simulink model "DIGITAL_WATCH_STAGE7"  (R2026b)
settings: Solver=VariableStepAuto  StopTime=3600
libraries: simulink_extras x21
settings Model: Creator=Trealer  LastModifiedBy=Trealer

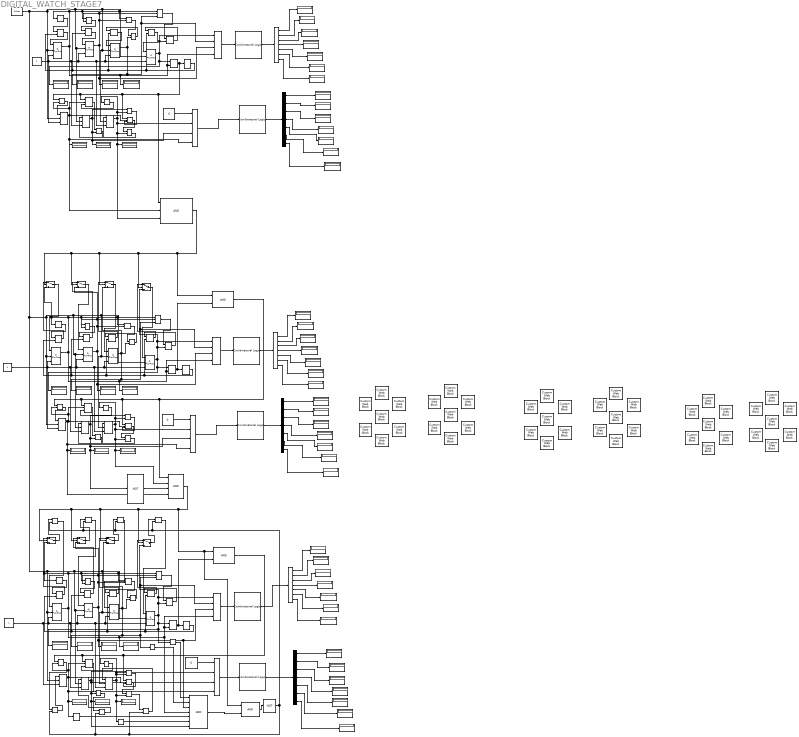
== system DIGITAL_WATCH_STAGE7 ==
  A{,1..5} (6 alike) : Display
  AND{,1..4,7..11,14,17..25} (20 alike) : Logic  IconShape=distinctive  AllPortsSameDT=off  OutDataTypeStr=boolean
  "AND-GATE MIN-EN " : Logic  Inputs=3  IconShape=distinctive  AllPortsSameDT=off  OutDataTypeStr=boolean
  AND-gate : Logic  IconShape=distinctive  AllPortsSameDT=off  OutDataTypeStr=boolean
  AND-gate1 : Logic  IconShape=distinctive  AllPortsSameDT=off  OutDataTypeStr=boolean
  AND-gate2 : Logic  Inputs=3  IconShape=distinctive  AllPortsSameDT=off  OutDataTypeStr=boolean
  AND-gate3 : Logic  Inputs=3  IconShape=distinctive  AllPortsSameDT=off  OutDataTypeStr=boolean
  AND-gate4 : Logic  IconShape=distinctive  AllPortsSameDT=off  OutDataTypeStr=boolean
  AND-gate5 : Logic  Inputs=3  IconShape=distinctive  AllPortsSameDT=off  OutDataTypeStr=boolean
  AND{5..6,12..13,15..16} (6 alike) : Logic  Inputs=3  IconShape=distinctive  AllPortsSameDT=off  OutDataTypeStr=boolean
  B{,1..5} (6 alike) : Display
  C{,1..5} (6 alike) : Display
  C_HR : Logic  IconShape=distinctive  AllPortsSameDT=off  OutDataTypeStr=boolean
  C_HU : Logic  IconShape=distinctive  AllPortsSameDT=off  OutDataTypeStr=boolean
  C_MIN : Logic  IconShape=distinctive  AllPortsSameDT=off  OutDataTypeStr=boolean
  C_MU : Logic  IconShape=distinctive  AllPortsSameDT=off  OutDataTypeStr=boolean
  Combinatorial Logic : CombinatorialLogic  TruthTable=|
      | [
      | 1 1 1 1 1 1 0;
      | 0 1 1 0 0 0 0;
      | 1 1 0 1 1 0 1;
      | 1 1 1 1 0 0 1;
      | 0 1 1 0 0 1 1;
      | 1 0 1 1 0 1 1;
      | 1 0 1 1 1 1 1;
      | 1 1 1 0 0 0 0;
      | 1 1 1 1 1 1 1;
      | 1 1 1 1 0 1 1;
      | 0 0 0 0 0 0 0;
      | 0 0 0 0 0 0 0;
      | 0 0 0 0 0 0 0;
      | 0 0 0 0 0 0 0;
      | 0 0 0 0 0 0 0;
      | 0 0 0 0 0 0 0
      | ]
  Combinatorial Logic1 : CombinatorialLogic  TruthTable=|
      | [
      | 1 1 1 1 1 1 0;
      | 0 1 1 0 0 0 0;
      | 1 1 0 1 1 0 1;
      | 1 1 1 1 0 0 1;
      | 0 1 1 0 0 1 1;
      | 1 0 1 1 0 1 1;
      | 1 0 1 1 1 1 1;
      | 1 1 1 0 0 0 0;
      | 1 1 1 1 1 1 1;
      | 1 1 1 1 0 1 1;
      | 0 0 0 0 0 0 0;
      | 0 0 0 0 0 0 0;
      | 0 0 0 0 0 0 0;
      | 0 0 0 0 0 0 0;
      | 0 0 0 0 0 0 0;
      | 0 0 0 0 0 0 0
      | ]
  Combinatorial Logic2 : CombinatorialLogic  TruthTable=|
      | [
      | 1 1 1 1 1 1 0;
      | 0 1 1 0 0 0 0;
      | 1 1 0 1 1 0 1;
      | 1 1 1 1 0 0 1;
      | 0 1 1 0 0 1 1;
      | 1 0 1 1 0 1 1;
      | 1 0 1 1 1 1 1;
      | 1 1 1 0 0 0 0;
      | 1 1 1 1 1 1 1;
      | 1 1 1 1 0 1 1;
      | 0 0 0 0 0 0 0;
      | 0 0 0 0 0 0 0;
      | 0 0 0 0 0 0 0;
      | 0 0 0 0 0 0 0;
      | 0 0 0 0 0 0 0;
      | 0 0 0 0 0 0 0
      | ]
  Combinatorial Logic3 : CombinatorialLogic  TruthTable=|
      | [
      | 1 1 1 1 1 1 0;
      | 0 1 1 0 0 0 0;
      | 1 1 0 1 1 0 1;
      | 1 1 1 1 0 0 1;
      | 0 1 1 0 0 1 1;
      | 1 0 1 1 0 1 1;
      | 1 0 1 1 1 1 1;
      | 1 1 1 0 0 0 0;
      | 1 1 1 1 1 1 1;
      | 1 1 1 1 0 1 1;
      | 0 0 0 0 0 0 0;
      | 0 0 0 0 0 0 0;
      | 0 0 0 0 0 0 0;
      | 0 0 0 0 0 0 0;
      | 0 0 0 0 0 0 0;
      | 0 0 0 0 0 0 0
      | ]
  Combinatorial Logic4 : CombinatorialLogic  TruthTable=|
      | [
      | 1 1 1 1 1 1 0;
      | 0 1 1 0 0 0 0;
      | 1 1 0 1 1 0 1;
      | 1 1 1 1 0 0 1;
      | 0 1 1 0 0 1 1;
      | 1 0 1 1 0 1 1;
      | 1 0 1 1 1 1 1;
      | 1 1 1 0 0 0 0;
      | 1 1 1 1 1 1 1;
      | 1 1 1 1 0 1 1;
      | 0 0 0 0 0 0 0;
      | 0 0 0 0 0 0 0;
      | 0 0 0 0 0 0 0;
      | 0 0 0 0 0 0 0;
      | 0 0 0 0 0 0 0;
      | 0 0 0 0 0 0 0
      | ]
  Combinatorial Logic5 : CombinatorialLogic  TruthTable=|
      | [
      | 1 1 1 1 1 1 0;
      | 0 1 1 0 0 0 0;
      | 1 1 0 1 1 0 1;
      | 1 1 1 1 0 0 1;
      | 0 1 1 0 0 1 1;
      | 1 0 1 1 0 1 1;
      | 1 0 1 1 1 1 1;
      | 1 1 1 0 0 0 0;
      | 1 1 1 1 1 1 1;
      | 1 1 1 1 0 1 1;
      | 0 0 0 0 0 0 0;
      | 0 0 0 0 0 0 0;
      | 0 0 0 0 0 0 0;
      | 0 0 0 0 0 0 0;
      | 0 0 0 0 0 0 0;
      | 0 0 0 0 0 0 0
      | ]
  Constant : Constant  Value=0  OutDataTypeStr=boolean
  Constant 1 : Constant  OutDataTypeStr=boolean
  Constant 2 : Constant  OutDataTypeStr=boolean
  Constant 3 : Constant  OutDataTypeStr=boolean
  Constant1 : Constant  Value=0  OutDataTypeStr=boolean
  Constant2 : Constant  Value=0  OutDataTypeStr=boolean
  D{,1..5} (6 alike) : Display
  Demux{,1..5} (6 alike) : Demux  Outputs=7
  Display{,1..8} (9 alike) : Display
  E{,1..5} (6 alike) : Display
  E_HU : Logic  Operator=NOT  IconShape=distinctive  AllPortsSameDT=off  OutDataTypeStr=boolean
  E_MIN : Logic  Operator=NOT  IconShape=distinctive  AllPortsSameDT=off  OutDataTypeStr=boolean
  F{,1..5} (6 alike) : Display
  G{,1..5} (6 alike) : Display
  HT0 : simulink_extras/Flip Flops/D Flip-Flop
  HT1 : simulink_extras/Flip Flops/D Flip-Flop
  HT2 : simulink_extras/Flip Flops/D Flip-Flop
  HU{0..3} (4 alike) : simulink_extras/Flip Flops/D Flip-Flop
  H_EN : Logic  Inputs=4  IconShape=distinctive  AllPortsSameDT=off  OutDataTypeStr=boolean
  H_RESET : Logic  IconShape=distinctive  AllPortsSameDT=off  OutDataTypeStr=boolean
  H_RUN : Logic  Operator=NOT  IconShape=distinctive  AllPortsSameDT=off  OutDataTypeStr=boolean
  Lamp{,1..41} (42 alike) : CustomWebBlock  LabelPosition=Hide  ShowInitialText=on  Configuration="{\"components\":[{\"name\":\"BackgroundImageComponent\",\"settings\":{\"image\":{\"size\":[150,150],\"src\":\"data:image\\/svg+xml;base64,PHN2ZyB4bWxucz0iaHR0cDovL3d3dy53My5vcmcvMjAwMC9zdmciIHhtbG5zOnhsaW5rPSJodHRwOi8vd3d3LnczLm9yZy8xOTk5L3hsaW5rIiB2aWV3Qm94PSIwIDAgNTAwIDUwMCI+PGRlZnM+PHN0eWxlPi5he2ZpbGw6dXJsKCNhKTt9LmJ7ZmlsbDp1cmwoI2IpO30uY3tmaWxsOnVybCgjYyk7fTwvc3R5bGU+PHJhZGlhbEdyYWRpZW50IGlkPSJhIiBjeD0iMjgzLjg0IiBjeT0iLTQ2Ni4zNyIgcj0iMzc1Ljc1IiBncmFkaWVudFRyYW5zZm9ybT0ibWF0cml4KDEuMzksIDAsIDAsIC0xLjM5LCAtMTUzLjU2LCAtNjQ0LjA4KSIg ...(+2088 chars)\",\"srcOrientation\":\"Right\"},\"position\":[0,0,1,1],\"scaleMode\":\"0\"}},{\"name\":\"LampStateComponent\",\"settings\":{\"position\":[0,0,1,1],\"states\":[{\"icon\":{\"customSrc\":\"data:image\\/svg+xml;base64,PHN2ZyBpZD0iTGF5ZXJfMSIgZGF0YS1uYW1lPSJMYXllciAxIiB4bWxucz0iaHR0cDovL3d3dy53My5vcmcvMjAwMC9zdmciIHZpZXdCb3g9IjAgMCA0MTEgNDU4Ij48ZGVmcz48c3R5bGU+LmNscy0xe2ZpbGw6I2ZkZjhjMTt9LmNscy0ye2ZpbGw6I2ZlZTEwMDt9LmNscy0ze2ZpbGw6IzIzMWYyMDt9LmNscy00e2ZpbGw6I2EwOWY5Zjt9LmNscy00LC5jbHMtNSwuY2xzLTZ7c3Ryb2tlOiMyMzFmMjA7c3Ryb2tlLW1pdGVybGltaXQ6MTA7fS5jbHMtNXtmaWxsOiNmZmY7fS5jbHMtNntmaWxsOm5vbmU7fTwvc3R5bGU+PC9kZWZz ...(+5168 chars)\",\"id\":-1,\"srcOrientation\":\"Right\",\"type\":\"custom\"},\"iconScale\":0.8,\"metadata\":{},\"overlayType\":\"intersect\",\"shape\":{\"color\":[0.725,0,0],\"opacity\":1,\"position\":[0.1,0.1,0.8,0.8],\"type\":\"ellipse\"},\"value\":[]},{\"icon\":{\"customSrc\":\"data:image\\/svg+xml;base64,PHN2ZyBpZD0iTGF5ZXJfMSIgZGF0YS1uYW1lPSJMYXllciAxIiB4bWxucz0iaHR0cDovL3d3dy53My5vcmcvMjAwMC9zdmciIHZpZXdCb3g9IjAgMCA0MTEgNDU4Ij48ZGVmcz48c3R5bGU+LmNscy0xe2ZpbGw6I2ZkZjhjMTt9LmNscy0ye2ZpbGw6I2ZlZTEwMDt9LmNscy0ze2ZpbGw6IzIzMWYyMDt9LmNscy00e2ZpbGw6I2EwOWY5Zjt9LmNscy00LC5jbHMtNSwuY2xzLTZ7c3Ryb2tlOiMyMzFmMjA7c3Ryb2tlLW1pdGVybGltaXQ6MTA7fS5jbHMtNXtmaWxsOiNmZmY7fS5jbHMtNntmaWxsOm5vbmU7fTwvc3R5bGU+PC9kZWZz ...(+5168 chars)\",\"id\":-1,\"srcOrientation\":\"Right\",\"type\":\"custom\"},\"iconScale\":0.8,\"metadata\":{\"useDefaults\":{\"customIcon\":true,\"icon\":true,\"overlayType\":true,\"shape\":true,\"sizeAndPosition\":true}},\"overlayType\":\"intersect\",\"shape\":{\"color\":[0,0,0],\"opacity\":1,\"position\":[0.1,0.1,0.8,0.8],\"type\":\"ellipse\"},\"value\":\"0\"},{\"icon\":{\"customSrc\":\"data:image\\/svg+xml;base64,PHN2ZyBpZD0iTGF5ZXJfMSIgZGF0YS1uYW1lPSJMYXllciAxIiB4bWxucz0iaHR0cDovL3d3dy53My5vcmcvMjAwMC9zdmciIHZpZXdCb3g9IjAgMCA0MTEgNDU4Ij48ZGVmcz48c3R5bGU+LmNscy0xe2ZpbGw6I2ZkZjhjMTt9LmNscy0ye2ZpbGw6I2ZlZTEwMDt9LmNscy0ze2ZpbGw6IzIzMWYyMDt9LmNscy00e2ZpbGw6I2EwOWY5Zjt9LmNscy00LC5jbHMtNSwuY2xzLTZ7c3Ryb2tlOiMyMzFmMjA7c3Ryb2tlLW1pdGVybGltaXQ6MTA7fS5jbHMtNXtmaWxsOiNmZmY7fS5jbHMtNntmaWxsOm5vbmU7fTwvc3R5bGU+PC9kZWZz ...(+5168 chars)\",\"id\":-1,\"srcOrientation\":\"Right\",\"type\":\"custom\"},\"iconScale\":0.8,\"metadata\":{\"useDefaults\":{\"customIcon\":true,\"icon\":true,\"overlayType\":true,\"shape\":true,\"sizeAndPosition\":true}},\"overlayType\":\"intersect\",\"shape\":{\"color\":[0,1,0],\"opacity\":1,\"position\":[0.1,0.1,0.8,0.8],\"type\":\"ellipse\"},\"value\":\"1\"}],\"valueType\":\"discrete\"}},{\"name\":\"ForegroundImageComponent\",\"settings\":{\"image\":{\"size\":[150,150],\"src\":\"data:image\\/svg+xml;base64,PHN2ZyB4bWxucz0iaHR0cDovL3d3dy53My5vcmcvMjAwMC9zdmciIHhtbG5zOnhsaW5rPSJodHRwOi8vd3d3LnczLm9yZy8xOTk5L3hsaW5rIiB2aWV3Qm94PSIwIDAgNTAwIDUwMCI+PGRlZnM+PHN0eWxlPi5he2ZpbGw6dXJsKCNhKTt9PC9zdHlsZT48bGluZWFyR3JhZGllbnQgaWQ9ImEiIHgxPSIxNzMuMDUiIHkxPSItNjI3Ljc4IiB4Mj0iMTczLjA1IiB5Mj0iLTUyMi40MyIgZ3JhZGllbnRUcmFuc2Zvcm09Im1hdHJpeCgxLjI5LCAwLCAwLCAtMS4zMywgMjcuMTMsIC02MjguMzEpIiBncmFkaWVudFVuaXRzPSJ1c2VyU3BhY2VPblVzZSI+PHN0b3Agb2Zmc2V0PSIwIiBzdG9wLWNvbG9yPSIjZmZmIiBzdG9wLW9wYWNpdHk9IjAuMjUiLz48c3RvcCBvZmZzZXQ9IjEiIHN0b3AtY29sb3I9IiNmZmYiIHN0b3Atb3BhY2l0eT0iMCIvPjwvbGluZWFyR3JhZGllbnQ+PC9kZWZzPjxwYXRoIGNsYXNzPSJhIiBkPSJNNDI5LjMsMTkwLjY2QzQwMi40NSwxMTQuNTEsMzMyLjY3LDYwLjE3LDI1MC44NSw2MC4xN2MtODMuNDMsMC0xNTQuMjgsNTYuNDItMTc5Ljk1LDEzNSwxNS4zNCwzOSw4OC4xMSw3LDE3Ny4wNyw3QzM0MCwyMDIuMDgsNDE3LjI2LDIzNi40Niw0MjkuMywxOTAuNjZaIi8+PC9zdmc+\",\"srcOrientation\":\"Right\"},\"isForeground\":1,\"position\":[0,0,1,1],\"scaleMode\":\"0\"}}],\"derived\":{\"blockParameters\":{\"CustomIcon\":\"data:image\\/svg+xml;base64,PHN2ZyBpZD0iTGF5ZXJfMSIgZGF0YS1uYW1lPSJMYXllciAxIiB4bWxucz0iaHR0cDovL3d3dy53My5vcmcvMjAwMC9zdmciIHZpZXdCb3g9IjAgMCA0MTEgNDU4Ij48ZGVmcz48c3R5bGU+LmNscy0xe2ZpbGw6I2ZkZjhjMTt9LmNscy0ye2ZpbGw6I2ZlZTEwMDt9LmNscy0ze2ZpbGw6IzIzMWYyMDt9LmNscy00e2ZpbGw6I2EwOWY5Zjt9LmNscy00LC5jbHMtNSwuY2xzLTZ7c3Ryb2tlOiMyMzFmMjA7c3Ryb2tlLW1pdGVybGltaXQ6MTA7fS5jbHMtNXtmaWxsOiNmZmY7fS5jbHMtNntmaWxsOm5vbmU7fTwvc3R5bGU+PC9kZWZz ...(+5168 chars)\",\"DefaultColor\":[0.725,0,0],\"Icon\":\"Custom\",\"StateColors\":[{\"color\":[0,0,0],\"value\":\"0\"},{\"color\":[0,1,0],\"value\":\"1\"}],\"StateValueType\":\"discrete\",\"fixedAspectRatio\":\"on\"}},\"settings\":{\"BindingType\":\"signal\",\"aspectRatio\":1.032258064516129,\"backgroundColor\":[0,0,0],\"backgroundOffset\":0.14,\"backgroundOpacity\":1,\"blockOrientation\":\"Right\",\"fixedAspectRatio\":\"on\",\"showBackgroundColor\":false,\"value\":0,\"version\":\"R2023a\"},\"type\":\"Lamp\"}"
  MT0 : simulink_extras/Flip Flops/D Flip-Flop
  MT1 : simulink_extras/Flip Flops/D Flip-Flop
  MT2 : simulink_extras/Flip Flops/D Flip-Flop
  MU{0..3} (4 alike) : simulink_extras/Flip Flops/D Flip-Flop
  Mux{,1..5} (6 alike) : Mux
  NOT{,1..8} (9 alike) : Logic  Operator=NOT  IconShape=distinctive  AllPortsSameDT=off  OutDataTypeStr=boolean
  NOT-gate : Logic  Operator=NOT  IconShape=distinctive  AllPortsSameDT=off  OutDataTypeStr=boolean
  NOT-gate1 : Logic  Operator=NOT  IconShape=distinctive  AllPortsSameDT=off  OutDataTypeStr=boolean
  NOT-gate2 : Logic  Operator=NOT  IconShape=distinctive  AllPortsSameDT=off  OutDataTypeStr=boolean
  OR : Logic  Operator=OR  IconShape=distinctive  AllPortsSameDT=off  OutDataTypeStr=boolean
  OR1 : Logic  Operator=OR  IconShape=distinctive  AllPortsSameDT=off  OutDataTypeStr=boolean
  OR2 : Logic  Operator=OR  IconShape=distinctive  AllPortsSameDT=off  OutDataTypeStr=boolean
  PULSE GENERATOR : DiscretePulseGenerator  PulseType=Time based  Period=1  PulseWidth=50
  Q{0..3} (4 alike) : simulink_extras/Flip Flops/D Flip-Flop
  Q0-Display : Display
  Q0-Display1 : Display
  Q0-Display2 : Display
  Q1-Display : Display
  Q1-Display1 : Display
  Q1-Display2 : Display
  Q2-Display : Display
  Q2-Display1 : Display
  Q2-Display2 : Display
  Q3-Display : Display
  Q3-Display1 : Display
  Q3-Display2 : Display
  R23 : Logic  Inputs=7  IconShape=distinctive  AllPortsSameDT=off  OutDataTypeStr=boolean
  Switch-{0..7} (8 alike) : Switch  Criteria=u2 ~= 0  SaturateOnIntegerOverflow=off  InputSameDT=off
  T0 : simulink_extras/Flip Flops/D Flip-Flop
  T1 : simulink_extras/Flip Flops/D Flip-Flop
  T2 : simulink_extras/Flip Flops/D Flip-Flop
  XOR{,1..8} (9 alike) : Logic  Operator=XOR  IconShape=distinctive  AllPortsSameDT=off  OutDataTypeStr=boolean
  XOR-gate{,1..8} (9 alike) : Logic  Operator=XOR  IconShape=distinctive  AllPortsSameDT=off  OutDataTypeStr=boolean
  wires:
  Constant 1/1 -> T1/3, T2/3, Q3/3, Q2/3, Q1/3, Q0/3, T0/3
  Q0/1 -> Mux/4, AND/2, Q0-Display/1, AND-gate/1, AND-gate2/1, XOR-gate/1, NOT-gate/1
  Q1/1 -> Mux/3, Q1-Display/1, AND-gate2/2, XOR-gate/2, AND-gate/2
  AND-gate/1 -> XOR-gate2/1
  Q2/1 -> Mux/2, AND-gate2/3, Q2-Display/1, XOR-gate2/2
  AND-gate2/1 -> XOR-gate3/1
  Q3/1 -> XOR-gate3/2, Mux/1, Q3-Display/1, AND/1
  AND/1 -> "AND-GATE MIN-EN "/1, AND6/1, AND5/1, XOR/1, NOT/1
  NOT-gate/1 -> AND1/1
  XOR-gate/1 -> AND2/1
  XOR-gate2/1 -> AND3/1
  XOR-gate3/1 -> AND4/1
  AND1/1 -> Q0/1
  AND2/1 -> Q1/1
  AND3/1 -> Q2/1
  AND4/1 -> Q3/1
  NOT/1 -> AND4/2, AND3/2, AND1/2, AND2/2
  T0/1 -> Display/1, Mux1/4, "AND-GATE MIN-EN "/2, AND6/2, AND5/2, XOR/2
  XOR/1 -> T0/1
  T2/1 -> "AND-GATE MIN-EN "/3, Display2/1, XOR2/2, Mux1/2, OR/2, NOT1/1
  NOT1/1 -> AND5/3
  AND5/1 -> XOR1/1
  T1/1 -> Mux1/3, Display1/1, XOR1/2, OR/1
  OR/1 -> AND6/3
  AND6/1 -> XOR2/1
  XOR1/1 -> T1/1
  XOR2/1 -> T2/1
  Mux/1 -> Combinatorial Logic/1
  Combinatorial Logic/1 -> Demux/1
  Demux/1 -> A/1
  Demux/2 -> B/1
  Demux/3 -> C/1
  Demux/4 -> D/1
  Demux/5 -> E/1
  Demux/6 -> F/1
  Demux/7 -> G/1
  Combinatorial Logic1/1 -> Demux1/1
  Constant/1 -> Mux1/1
  Mux1/1 -> Combinatorial Logic1/1
  Demux1/2 -> B1/1
  Demux1/6 -> F1/1
  Demux1/1 -> A1/1
  Demux1/7 -> G1/1
  Demux1/4 -> D1/1
  Demux1/3 -> C1/1
  Demux1/5 -> E1/1
  Demux3/2 -> B3/1
  Demux3/4 -> D3/1
  Demux3/3 -> C3/1
  Demux3/7 -> G3/1
  Constant1/1 -> Mux3/1
  Demux3/5 -> E3/1
  Demux3/1 -> A3/1
  Combinatorial Logic3/1 -> Demux3/1
  MU3/1 -> Switch-3/3, Mux2/1, XOR-gate5/2, Q3-Display1/1, C_MU/1
  XOR-gate1/1 -> AND9/1
  NOT-gate1/1 -> AND8/1
  Demux2/3 -> C2/1
  XOR-gate4/1 -> AND10/1
  C_MU/1 -> C_MIN/2, E_MIN/1
  NOT3/1 -> AND12/3
  XOR5/1 -> MT2/1
  XOR3/1 -> MT0/1
  MU2/1 -> XOR-gate4/2, Mux2/2, AND-gate3/3, Q2-Display1/1, Switch-2/3
  AND-gate1/1 -> XOR-gate4/1
  XOR-gate5/1 -> AND11/1
  Demux2/2 -> B2/1
  Demux2/1 -> A2/1
  Combinatorial Logic2/1 -> Demux2/1
  Demux2/7 -> G2/1
  OR1/1 -> AND13/3
  MU0/1 -> AND-gate1/1, AND-gate3/1, XOR-gate1/1, Switch-0/3, NOT-gate1/1, Mux2/4, C_MU/2, Q0-Display1/1
  E_MIN/1 -> AND11/2, AND10/2, AND8/2, AND9/2
  Constant 2/1 -> MT1/3, MT2/3, MU3/3, MU2/3, MU1/3, MU0/3, MT0/3
  Demux2/4 -> D2/1
  MU1/1 -> Switch-1/3, AND-gate3/2, XOR-gate1/2, AND-gate1/2, Mux2/3, Q1-Display1/1
  Demux2/5 -> E2/1
  Mux3/1 -> Combinatorial Logic3/1
  Demux2/6 -> F2/1
  AND13/1 -> XOR5/1
  MT0/1 -> H_EN/4, Display3/1, Mux3/4, AND12/2, XOR3/2, AND13/2
  AND-gate3/1 -> XOR-gate5/1
  AND12/1 -> XOR4/1
  XOR4/1 -> MT1/1
  Mux2/1 -> Combinatorial Logic2/1
  MT2/1 -> H_EN/2, Display5/1, XOR5/2, Mux3/2, OR1/2, NOT3/1
  Demux3/6 -> F3/1
  MT1/1 -> NOT4/1, Display4/1, Mux3/3, XOR4/2, OR1/1
  "AND-GATE MIN-EN "/1 -> C_MIN/1, Switch-3/2, Switch-2/2, Switch-1/2, Switch-0/2
  AND8/1 -> Switch-0/1
  Switch-0/1 -> MU0/1
  AND9/1 -> Switch-1/1
  Switch-1/1 -> MU1/1
  AND10/1 -> Switch-2/1
  Switch-2/1 -> MU2/1
  AND11/1 -> Switch-3/1
  Switch-3/1 -> MU3/1
  C_MIN/1 -> H_EN/1, AND13/1, AND12/1, XOR3/1
  NOT4/1 -> H_EN/3
  PULSE GENERATOR/1 -> HU3/2, HT2/2, HU2/2, HU1/2, HT1/2, HT0/2, HU0/2, MU3/2, MT2/2, MU2/2, MU1/2, MT1/2, MU0/2, MT0/2, Q3/2, T2/2, Q2/2, Q1/2, T1/2, Q0/2, T0/2
  AND17/1 -> Switch-4/1
  AND7/1 -> Switch-6/1
  HT1/1 -> R23/7, Display7/1, XOR7/2, Mux5/3, OR2/1
  Demux5/6 -> F5/1
  HT2/1 -> NOT6/1, Mux5/2, OR2/2, NOT5/1, Display8/1, XOR8/2
  AND15/1 -> XOR7/1
  AND-gate5/1 -> XOR-gate8/1
  AND16/1 -> XOR8/1
  Mux4/1 -> Combinatorial Logic4/1
  Demux4/6 -> F4/1
  HT0/1 -> NOT2/1, Display6/1, Mux5/4, AND15/2, XOR6/2, AND16/2
  Mux5/1 -> Combinatorial Logic5/1
  AND14/1 -> Switch-7/1
  C_HR/1 -> AND16/1, AND15/1, XOR6/1
  HU1/1 -> Switch-5/3, AND-gate5/2, XOR-gate6/2, AND-gate4/2, Mux4/3, R23/3, Q1-Display2/1
  Demux4/4 -> D4/1
  Constant 3/1 -> HT1/3, HT2/3, HU3/3, HU2/3, HU1/3, HU0/3, HT0/3
  E_HU/1 -> AND14/2, AND7/2, AND17/2, AND18/2
  HU0/1 -> R23/4, C_HU/2, Mux4/4, Q0-Display2/1, NOT-gate2/1, Switch-4/3, AND-gate4/1, AND-gate5/1, XOR-gate6/1
  OR2/1 -> AND16/3
  Combinatorial Logic4/1 -> Demux4/1
  Demux4/1 -> A4/1
  HU2/1 -> XOR-gate7/2, NOT7/1, Mux4/2, AND-gate5/3, Q2-Display2/1, Switch-6/3
  Demux4/7 -> G4/1
  XOR-gate8/1 -> AND14/1
  AND-gate4/1 -> XOR-gate7/1
  NOT6/1 -> AND15/3
  C_HU/1 -> C_HR/2, E_HU/1
  XOR-gate7/1 -> AND7/1
  Demux4/3 -> C4/1
  NOT-gate2/1 -> AND17/1
  HU3/1 -> Switch-7/3, Mux4/1, XOR-gate8/2, NOT8/1, Q3-Display2/1, C_HU/1
  AND18/1 -> Switch-5/1
  Combinatorial Logic5/1 -> Demux5/1
  Demux4/5 -> E4/1
  Demux4/2 -> B4/1
  Demux5/7 -> G5/1
  Demux5/3 -> C5/1
  Demux5/5 -> E5/1
  Demux5/1 -> A5/1
  Constant2/1 -> Mux5/1
  Demux5/2 -> B5/1
  Demux5/4 -> D5/1
  H_EN/1 -> C_HR/1, H_RESET/1, Switch-7/2, Switch-6/2, Switch-5/2, Switch-4/2
  XOR-gate6/1 -> AND18/1
  NOT2/1 -> R23/5
  NOT8/1 -> R23/1
  NOT7/1 -> R23/2
  NOT5/1 -> R23/6
  R23/1 -> H_RESET/2
  H_RESET/1 -> H_RUN/1
  H_RUN/1 -> AND25/2, AND24/2, AND23/2, AND22/2, AND21/2, AND20/2, AND19/2
  Switch-4/1 -> AND19/1
  AND19/1 -> HU0/1
  Switch-5/1 -> AND20/1
  AND20/1 -> HU1/1
  Switch-6/1 -> AND21/1
  AND21/1 -> HU2/1
  Switch-7/1 -> AND22/1
  AND22/1 -> HU3/1
  XOR6/1 -> AND23/1
  AND23/1 -> HT0/1
  XOR7/1 -> AND24/1
  AND24/1 -> HT1/1
  XOR8/1 -> AND25/1
  AND25/1 -> HT2/1
